simulink model "fir_mbd_float"  (R2026a)
settings: Solver=FixedStepDiscrete  StopTime=300  FixedStep=1
model workspace (MAT data in the model file):
  b = [0.125 0.375 0.375 0.125]
  f_noise = 0.4
  f_sig = 0.01
settings Model: Creator=KoayXianCong  LastModifiedBy=KoayXianCong

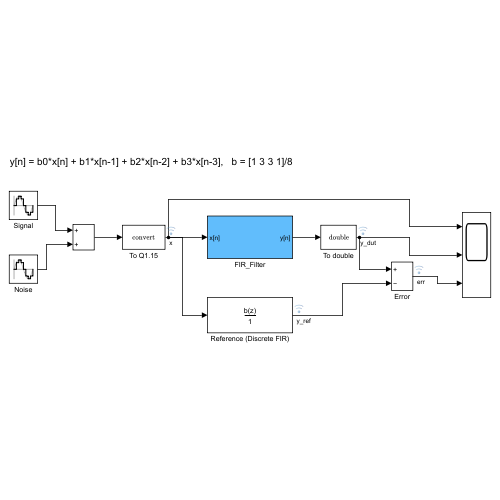
[thumbnail: Simulink's stored preview of the top-level diagram]
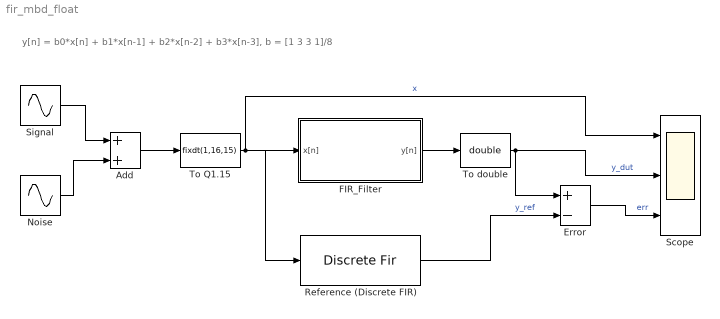
== system fir_mbd_float ==
  note: y[n] = b0*x[n] + b1*x[n-1] + b2*x[n-2] + b3*x[n-3], b = [1 3 3 1]/8
  Add : Sum
  Error : Sum  Inputs=+-
  FIR_Filter : Subsystem
  Noise : Sin  Amplitude=0.4  Frequency=2*pi*f_noise  SampleTime=1
  Reference (Discrete FIR) : DiscreteFir  Coefficients=b
  Scope : Scope  NumInputPorts=3
      settings: TimeSpan=300
  Signal : Sin  Amplitude=0.5  Frequency=2*pi*f_sig  SampleTime=1
  To Q1.15 : DataTypeConversion  OutDataTypeStr=fixdt(1,16,15)  RndMeth=Nearest
  To double : DataTypeConversion  OutDataTypeStr=double  SaturateOnIntegerOverflow=off  RndMeth=Floor
  wires:
  Signal/1 -> Add/1
  Noise/1 -> Add/2
  Add/1 -> To Q1.15/1
  To Q1.15/1 -> Reference (Discrete FIR)/1, Scope/1, FIR_Filter/1(x[n])  "x"
  FIR_Filter/1(y[n]) -> To double/1
  To double/1 -> Scope/2, Error/1  "y_dut"
  Reference (Discrete FIR)/1 -> Error/2  "y_ref"
  Error/1 -> Scope/3  "err"

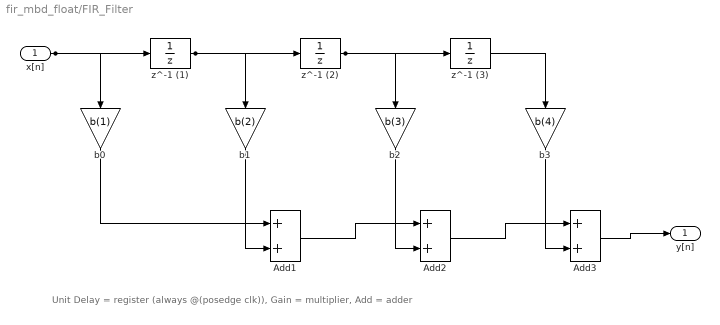
== system fir_mbd_float/FIR_Filter ==
  note: Unit Delay = register (always @(posedge clk)), Gain = multiplier, Add = adder
  x[n] : Inport
  Add1 : Sum  OutDataTypeStr=double
  Add2 : Sum  OutDataTypeStr=double
  Add3 : Sum  OutDataTypeStr=double
  b0 : Gain  Gain=b(1)  ParamDataTypeStr=double  OutDataTypeStr=double
  b1 : Gain  Gain=b(2)  ParamDataTypeStr=double  OutDataTypeStr=double
  b2 : Gain  Gain=b(3)  ParamDataTypeStr=double  OutDataTypeStr=double
  b3 : Gain  Gain=b(4)  ParamDataTypeStr=double  OutDataTypeStr=double
  z^-1 (1) : UnitDelay  SampleTime=-1
  z^-1 (2) : UnitDelay  SampleTime=-1
  z^-1 (3) : UnitDelay  SampleTime=-1
  y[n] : Outport
  wires:
  x[n]/1 -> z^-1 (1)/1, b0/1
  z^-1 (1)/1 -> z^-1 (2)/1, b1/1
  z^-1 (2)/1 -> z^-1 (3)/1, b2/1
  z^-1 (3)/1 -> b3/1
  b0/1 -> Add1/1
  b1/1 -> Add1/2
  Add1/1 -> Add2/1
  b2/1 -> Add2/2
  Add2/1 -> Add3/1
  b3/1 -> Add3/2
  Add3/1 -> y[n]/1
